simulink model "w6_stage4_3_held_pwm10k"  (R2026a)
settings: Solver=ode23t  StopTime=0.1  MaxStep=5e-06  RelTol=1e-6  AbsTol=1e-9
settings Model: Creator=cogml  LastModifiedBy=cogml

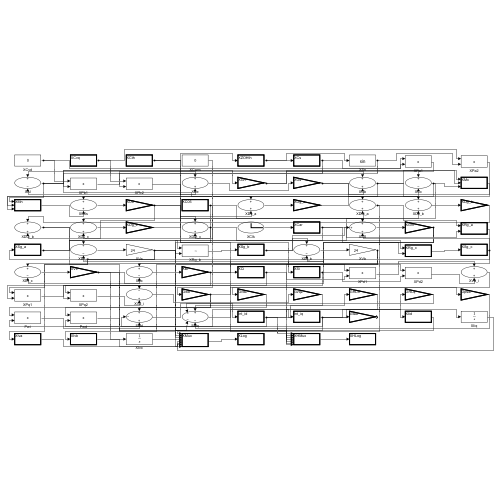
[thumbnail: Simulink's stored preview of the top-level diagram]
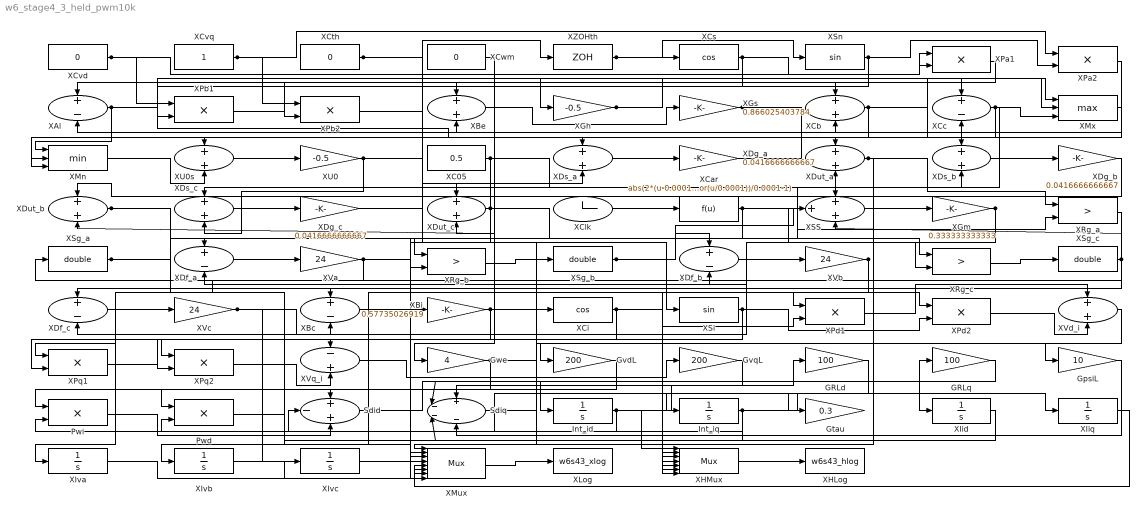
== system w6_stage4_3_held_pwm10k ==
  GRLd : Gain  Gain=100
  GRLq : Gain  Gain=100
  GpsiL : Gain  Gain=10
  Gtau : Gain  Gain=0.3
  GvdL : Gain  Gain=200
  GvqL : Gain  Gain=200
  Gwe : Gain  Gain=4
  Int_id : Integrator
  Int_iq : Integrator
  Pwd : Product
  Pwi : Product
  Sdid : Sum  Inputs=+-+
  Sdiq : Sum  Inputs=+---
  XAl : Sum  Inputs=+-
  XBc : Sum  Inputs=+-
  XBe : Sum
  XBi : Gain  Gain=0.57735026919
  XC05 : Constant  Value=0.5
  XCar : Fcn  Expr=abs(2*(u-0.0001*floor(u/0.0001))/0.0001-1)
  XCb : Sum
  XCc : Sum  Inputs=+-
  XCi : Trigonometry  Operator=cos
  XClk : Clock
  XCs : Trigonometry  Operator=cos
  XCth : Constant  Value=0
  XCvd : Constant  Value=0
  XCvq : Constant
  XCwm : Constant  Value=0
  XDf_a : Sum  Inputs=+-
  XDf_b : Sum  Inputs=+-
  XDf_c : Sum  Inputs=+-
  XDg_a : Gain  Gain=0.0416666666667
  XDg_b : Gain  Gain=0.0416666666667
  XDg_c : Gain  Gain=0.0416666666667
  XDs_a : Sum
  XDs_b : Sum
  XDs_c : Sum
  XDut_a : Sum
  XDut_b : Sum
  XDut_c : Sum
  XGh : Gain  Gain=-0.5
  XGm : Gain  Gain=0.333333333333
  XGs : Gain  Gain=0.866025403784
  XHLog : ToWorkspace  VariableName=w6s43_hlog  SaveFormat=Timeseries  SampleTime=-1
  XHMux : Mux  Inputs=7
  XIid : Integrator
  XIiq : Integrator
  XIva : Integrator
  XIvb : Integrator
  XIvc : Integrator
  XLog : ToWorkspace  VariableName=w6s43_xlog  SaveFormat=Timeseries  SampleTime=0.0001
  XMn : MinMax  Inputs=3
  XMux : Mux  Inputs=8
  XMx : MinMax  Function=max  Inputs=3
  XPa1 : Product
  XPa2 : Product
  XPb1 : Product
  XPb2 : Product
  XPd1 : Product
  XPd2 : Product
  XPq1 : Product
  XPq2 : Product
  XRg_a : RelationalOperator  Operator=>  OutDataTypeStr=boolean  RndMeth=Simplest  InputSameDT=off
  XRg_b : RelationalOperator  Operator=>  OutDataTypeStr=boolean  RndMeth=Simplest  InputSameDT=off
  XRg_c : RelationalOperator  Operator=>  OutDataTypeStr=boolean  RndMeth=Simplest  InputSameDT=off
  XSS : Sum  Inputs=+++
  XSg_a : DataTypeConversion  OutDataTypeStr=double  SaturateOnIntegerOverflow=off  RndMeth=Floor
  XSg_b : DataTypeConversion  OutDataTypeStr=double  SaturateOnIntegerOverflow=off  RndMeth=Floor
  XSg_c : DataTypeConversion  OutDataTypeStr=double  SaturateOnIntegerOverflow=off  RndMeth=Floor
  XSi : Trigonometry
  XSn : Trigonometry
  XU0 : Gain  Gain=-0.5
  XU0s : Sum
  XVa : Gain  Gain=24
  XVb : Gain  Gain=24
  XVc : Gain  Gain=24
  XVd_i : Sum
  XVq_i : Sum  Inputs=-+
  XZOHth : ZeroOrderHold  SampleTime=0.0001
  wires:
  XCth/1 -> XZOHth/1, XCi/1, XSi/1
  XZOHth/1 -> XCs/1, XSn/1
  XCvd/1 -> XPa1/1, XPb1/1
  XCs/1 -> XPa1/2, XPb2/2
  XCvq/1 -> XPa2/1, XPb2/1
  XSn/1 -> XPa2/2, XPb1/2
  XPa1/1 -> XAl/1
  XPa2/1 -> XAl/2
  XPb1/1 -> XBe/1
  XPb2/1 -> XBe/2
  XAl/1 -> XGh/1, XMx/1, XMn/1, XDs_a/1
  XBe/1 -> XGs/1
  XGh/1 -> XCb/1, XCc/1
  XGs/1 -> XCb/2, XCc/2
  XCb/1 -> XMx/2, XMn/2, XDs_b/1
  XCc/1 -> XMx/3, XMn/3, XDs_c/1
  XMx/1 -> XU0s/1
  XMn/1 -> XU0s/2
  XU0s/1 -> XU0/1
  XU0/1 -> XDs_a/2, XDs_b/2, XDs_c/2
  XDs_a/1 -> XDg_a/1
  XDg_a/1 -> XDut_a/1
  XC05/1 -> XDut_a/2, XDut_b/2, XDut_c/2
  XDs_b/1 -> XDg_b/1
  XDg_b/1 -> XDut_b/1
  XDs_c/1 -> XDg_c/1
  XDg_c/1 -> XDut_c/1
  XClk/1 -> XCar/1
  XDut_a/1 -> XRg_a/1, XMux/1
  XCar/1 -> XRg_a/2, XRg_b/2, XRg_c/2
  XRg_a/1 -> XSg_a/1
  XSg_a/1 -> XSS/1, XDf_a/1
  XDut_b/1 -> XRg_b/1, XMux/2
  XRg_b/1 -> XSg_b/1
  XSg_b/1 -> XSS/2, XDf_b/1
  XDut_c/1 -> XRg_c/1, XMux/3
  XRg_c/1 -> XSg_c/1
  XSg_c/1 -> XSS/3, XDf_c/1
  XSS/1 -> XGm/1
  XGm/1 -> XDf_a/2, XDf_b/2, XDf_c/2
  XDf_a/1 -> XVa/1
  XDf_b/1 -> XVb/1
  XDf_c/1 -> XVc/1
  XVb/1 -> XBc/1, XIvb/1, XHMux/6
  XVc/1 -> XBc/2, XIvc/1, XHMux/7
  XBc/1 -> XBi/1
  XVa/1 -> XPd1/1, XPq1/1, XIva/1, XHMux/3, XHMux/5
  XCi/1 -> XPd1/2, XPq2/2
  XBi/1 -> XPd2/1, XPq2/1, XHMux/4
  XSi/1 -> XPd2/2, XPq1/2
  XPd1/1 -> XVd_i/1
  XPd2/1 -> XVd_i/2
  XPq1/1 -> XVq_i/1
  XPq2/1 -> XVq_i/2
  XCwm/1 -> Gwe/1
  XVd_i/1 -> GvdL/1
  XVq_i/1 -> GvqL/1
  Int_id/1 -> GRLd/1, Pwd/2, XIid/1, XHMux/1
  Int_iq/1 -> GRLq/1, Pwi/2, Gtau/1, XIiq/1, XHMux/2
  Gwe/1 -> Pwi/1, Pwd/1, GpsiL/1
  GvdL/1 -> Sdid/1
  GRLd/1 -> Sdid/2
  Pwi/1 -> Sdid/3
  GvqL/1 -> Sdiq/1
  GRLq/1 -> Sdiq/2
  Pwd/1 -> Sdiq/3
  GpsiL/1 -> Sdiq/4
  Sdid/1 -> Int_id/1
  Sdiq/1 -> Int_iq/1
  XIid/1 -> XMux/4
  XIiq/1 -> XMux/5
  XIva/1 -> XMux/6
  XIvb/1 -> XMux/7
  XIvc/1 -> XMux/8
  XMux/1 -> XLog/1
  XHMux/1 -> XHLog/1
